simulink model "Transformer_Subsystem"  (R2025a)
settings: Solver=ode45  StartTime=0.0  StopTime=86400  MaxStep=1e-4  MinStep=1e-8  RelTol=1e-5  AbsTol=1e-8
settings Model: Creator=denis  LastModifiedBy=denis

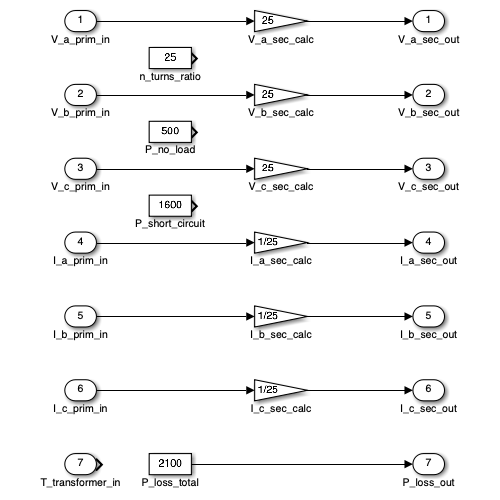
[thumbnail: Simulink's stored preview of the top-level diagram]
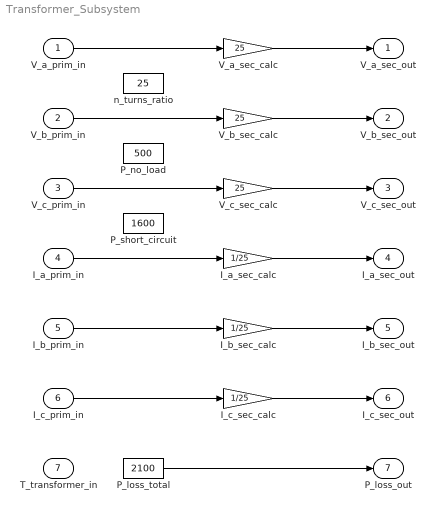
== system Transformer_Subsystem ==
  V_a_prim_in : Inport
  V_b_prim_in : Inport  Port=2
  V_c_prim_in : Inport  Port=3
  I_a_prim_in : Inport  Port=4
  I_b_prim_in : Inport  Port=5
  I_c_prim_in : Inport  Port=6
  T_transformer_in : Inport  Port=7
  I_a_sec_calc : Gain  Gain=1/25
  I_b_sec_calc : Gain  Gain=1/25
  I_c_sec_calc : Gain  Gain=1/25
  P_loss_total : Constant  Value=2100
  P_no_load : Constant  Value=500
  P_short_circuit : Constant  Value=1600
  V_a_sec_calc : Gain  Gain=25
  V_b_sec_calc : Gain  Gain=25
  V_c_sec_calc : Gain  Gain=25
  n_turns_ratio : Constant  Value=25
  V_a_sec_out : Outport
  V_b_sec_out : Outport  Port=2
  V_c_sec_out : Outport  Port=3
  I_a_sec_out : Outport  Port=4
  I_b_sec_out : Outport  Port=5
  I_c_sec_out : Outport  Port=6
  P_loss_out : Outport  Port=7
  wires:
  V_a_prim_in/1 -> V_a_sec_calc/1
  V_b_prim_in/1 -> V_b_sec_calc/1
  V_c_prim_in/1 -> V_c_sec_calc/1
  I_a_prim_in/1 -> I_a_sec_calc/1
  I_b_prim_in/1 -> I_b_sec_calc/1
  I_c_prim_in/1 -> I_c_sec_calc/1
  V_a_sec_calc/1 -> V_a_sec_out/1
  V_b_sec_calc/1 -> V_b_sec_out/1
  V_c_sec_calc/1 -> V_c_sec_out/1
  I_a_sec_calc/1 -> I_a_sec_out/1
  I_b_sec_calc/1 -> I_b_sec_out/1
  I_c_sec_calc/1 -> I_c_sec_out/1
  P_loss_total/1 -> P_loss_out/1
